simulink model "sldrtex_controller_3"  (R2015a)
settings: Solver=ode5  StartTime=0.0  StopTime=10.0  RelTol=1e-3
undefined symbols (not defined in the file): National_Instruments, PCI, sigbuilder_block
libraries: sldrtlib x1
Description:
  | Real-Time Controller
  | 
  | This model shows how to build a simple closed-loop real-time controller using
  | Simulink Desktop Real-Time. The output of the controlled plant is connected
  | to the analog input of your data acquisition board. This signal is subtracted from
  | the set point value generated by the signal generator and processed by a PID
  | controller. The output of the controller drives the input of the plant using the analog
  | output of your data acquisition board.
  | 
  | This model is a simplified version of the controller used for the CE152 Magnetic
  | Levitation Model.
  | 
  | How to run this model in Normal Mode:
  | 
  | 1) Open the Analog Input and Analog Output blocks and select your data acquisition
  |    board. If there's no board installed, install it using the Install new board button.
  | 2) Double-click the orange button to switch to Normal Mode if needed.
  | 3) Start the real-time execution using Simulation->Run.
  | 
  | How to run this model in External Mode:
  | 
  | 1) Open the Analog Input and Analog Output blocks and select your data acquisition
  |    board. If there's no board installed, install it using the Install new board button.
  | 2) Double-click the orange button to switch to External Mode if needed.
  | 3) Start the real-time execution using Simulation->Run. The model will automatically
  |    build, connect to Simulink in External Mode and start.
  | 
  | Note:
  | To run this model, you must have a data acquisition board connected to your
  |    computer.
settings Model: CovSFcnEnable=off  ExtModeTrigDuration=10000  Creator=The MathWorks Inc.  LastModifiedBy=Aluno-05
settings DataIOCC: SignalLoggingName=logsOut
settings OptimizationCC: ExpressionDepthLimit=2147483647  InitFltsAndDblsToZero=on  EfficientMapNaN2IntZero=off
settings DebuggingCC: UnderspecifiedInitializationDetection=Classic  MergeDetectMultiDrivingBlocksExec=none  SignalResolutionControl=TryResolveAllWithWarning  FcnCallInpInsideContextMsg=UseLocalSettings  StateNameClashWarn=warning
settings HardwareCC: ProdBitPerLong=64  ProdBitPerPointer=64  ProdIntDivRoundTo=Zero  ProdEndianess=LittleEndian  ProdWordSize=64  ProdHWDeviceType=Intel->x86-64  TargetBitPerLong=64  TargetBitPerPointer=64  TargetIntDivRoundTo=Zero  TargetEndianess=LittleEndian  TargetWordSize=64  TargetHWDeviceType=Intel->x86-64
settings RTWCC: SystemTargetFile=rtwin.tlc  TemplateMakefile=rtwin.tmf  Description=Simulink Desktop Real-Time
settings RTWinTargetCC: TargetPreCompLibLocation=C:\Program Files\MATLAB\MATLAB Production Server\R2015a\toolbox\sldrt\lib\win64

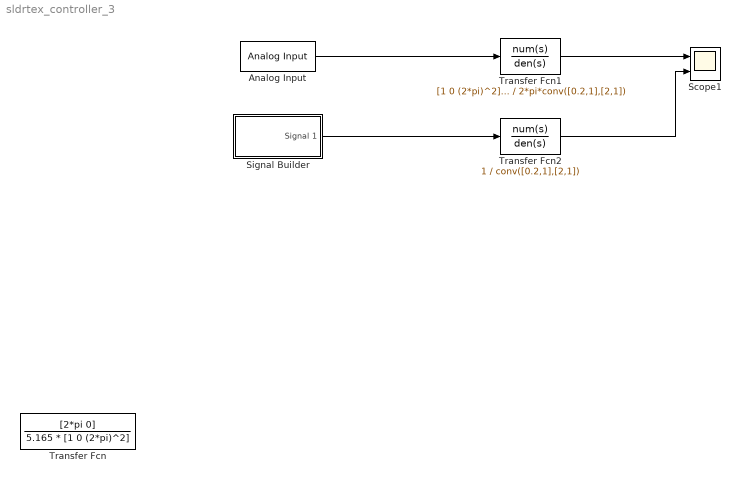
== system sldrtex_controller_3 ==
  Analog Input : sldrtlib/Analog Input  SampleTime=10e-3  MaxMissedTicks=20  ShowMissedTicks=off  YieldWhenWaiting=off  DrvName=National_Instruments/PCI-6221  DrvAddress=4294967295  DrvOptions=[0 0 0 0 0]  Channels=1  RangeMode=1  VoltRange=1  DataType=1
      settings: AttributesFormatString=National Instruments\nPCI-6221 [auto]
  Scope1 : Scope  NumInputPorts=2
      settings: TimeRange=10  YMin=0.05~0  YMax=0.375~0.00025  MaxDataPoints=10000  SampleInput=on  SampleTime=10e-3
  Signal Builder : Subsystem  Tag=STV Subsys  LoadFcn=sigbuilder_block('load');  StartFcn=sigbuilder_block('start');  StopFcn=sigbuilder_block('stop');  ClipboardFcn=sigbuilder_block('clipboard');  mask(Sigbuilder block){}
      mask help: Simulink:masks:SigbuilderBlock_MD
      mask init:
      | if ~strcmp(get_param(bdroot(gcbh),'SimulationStatus'),'stopped') tuvar = sigbuilder_block('maskInit'); end
      settings: CopyFcn=sigbuilder_block('copy');  DeleteFcn=sigbuilder_block('delete');  ModelCloseFcn=sigbuilder_block('modelClose');  PreSaveFcn=sigbuilder_block('preSave');  PauseFcn=sigbuilder_block('pause');  ContinueFcn=sigbuilder_block('continue');  NameChangeFcn=sigbuilder_block('namechange');  OpenFcn=sigbuilder_block('open',[437.6 199.2 550.4 400 ]);  CloseFcn=sigbuilder_block('close');
      mask Display: plot(0, 0, 100, 100,[2, 2, 32, 32, 2], [68, 8, 8, 68, 68],[32, 2], [38, 38], [32, 19, 2],[53, 60, 44], [32, 17, 17, 2],[16, 16, 31, 31]);txt = getActiveGroup(gcbh);text(2, 100, txt,'verticalAlignment', 'top');
  Transfer Fcn : TransferFcn  Numerator=[2*pi 0]  Denominator=5.165 * [1 0 (2*pi)^2]
  Transfer Fcn1 : TransferFcn  Numerator=[1 0 (2*pi)^2]  Denominator=2*pi*conv([0.2,1],[2,1])
  Transfer Fcn2 : TransferFcn  Numerator=1  Denominator=conv([0.2,1],[2,1])
  wires:
  Analog Input/1 -> Transfer Fcn1/1
  Transfer Fcn1/1 -> Scope1/1
  Transfer Fcn2/1 -> Scope1/2
  Signal Builder/1(Signal 1) -> Transfer Fcn2/1

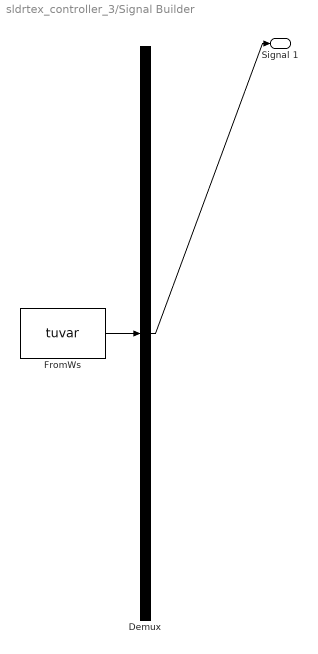
== system sldrtex_controller_3/Signal Builder ==
  Demux : Demux  Tag=STV Demux  Outputs=1
  FromWs : FromWorkspace  Tag=STV FromWs  VariableName=tuvar  SampleTime=0
      SigBuilderData=|
      | common.afterFinalStr = 'Extrapolate'
      | common.sampleTime = 0
      | dataSet.timeRange = [0 10]
      | dataSet.name = 'Group 1'
      | sbobj.Groups.Name = 'Group 1'
      | sbobj.Groups.Signals.Name = 'Signal 1'
      | sbobj.Groups.Signals.XData = [0 1e-10 1e-10 10]
      | sbobj.Groups.Signals.YData = [1 1 0 0]
  Signal 1 : Outport  Tag=STV Outport
  wires:
  FromWs/1 -> Demux/1
  Demux/1 -> Signal 1/1
